simulink model "MPCFSCRL"  (R2024a)
settings: Solver=VariableStepAuto  StartTime=0.0  StopTime=0.04  RelTol=1e-3
values from neighbouring files (symbols this model uses):
  A = (2/3)*[1 -1/2 -1/2; 0 sqrt(3)/2 -sqrt(3)/2]    [AgenteRL.m]
  C = 1000e-6    (= 0.001)    [AgenteRL.m]
  Ls = 10e-3    (= 0.01)    [AgenteRL.m]
  R = 0.1    [AgenteRL.m]
  Rs = 0.1    [AgenteRL.m]
  Ts = 10e-6    (= 1e-05)    [AgenteRL.m]
  Vcc = 350    [AgenteRL.m]
  Vg = 110    [AgenteRL.m]
libraries: spsSeriesRLCBranchLib x5, spsACVoltageSourceLib x3, spsThreePhaseVIMeasurementLib x2, rllib x1, spsDCVoltageSourceLib x1, spsGroundLib x1, spsUniversalBridgeLib x1, spsVoltageMeasurementLib x1, spspowerguiLib x1
settings Model: Creator=nalv_  LastModifiedBy=Raphael Teixeira

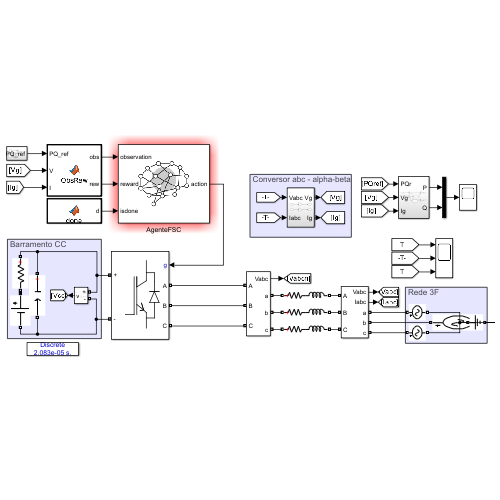
[thumbnail: Simulink's stored preview of the top-level diagram]
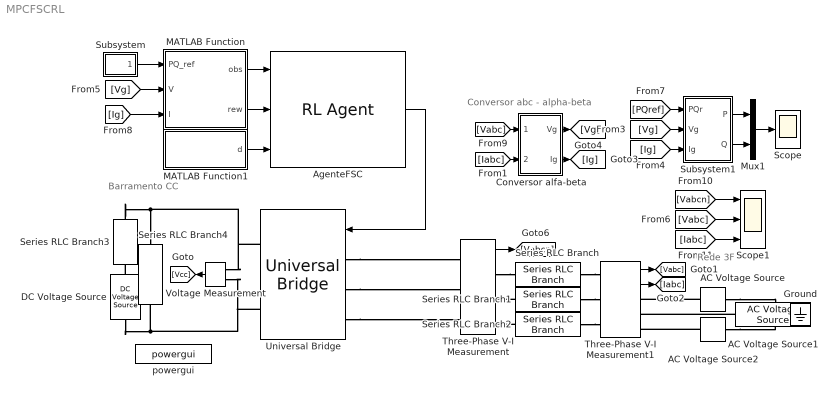
== system MPCFSCRL ==
  note: Barramento CC
  note: Conversor abc - alpha-beta
  note: Rede 3F
  AC Voltage Source : spsACVoltageSourceLib/AC Voltage Source  Amplitude=Vg  Phase=0  Frequency=60  SampleTime=Ts  Measurements=None  BusType=swing  Pref=10e3  Qref=0  Qmin=-inf  Qmax=+inf
  AC Voltage Source1 : spsACVoltageSourceLib/AC Voltage Source  Amplitude=Vg  Phase=120  Frequency=60  SampleTime=Ts  Measurements=None  BusType=swing  Pref=10e3  Qref=0  Qmin=-inf  Qmax=+inf
  AC Voltage Source2 : spsACVoltageSourceLib/AC Voltage Source  Amplitude=Vg  Phase=-120  Frequency=60  SampleTime=Ts  Measurements=None  BusType=swing  Pref=10e3  Qref=0  Qmin=-inf  Qmax=+inf
  AgenteFSC : rllib/RL Agent  Agent=agentObj  ExternalActionAsInput=off  ProvideLastAction=off  ProvideCumRwd=off  TreatAsDirectFeedthrough=on  UseStrictObservationDataTypes=off
  Conversor alfa-beta : Subsystem
  DC Voltage Source : spsDCVoltageSourceLib/DC Voltage Source  Amplitude=Vcc  Measurements=None
  Ground : spsGroundLib/Ground  LConnTagsString=a
  MATLAB Function : MATLAB Function  TreatAsAtomicUnit=on
  MATLAB Function1 : MATLAB Function  TreatAsAtomicUnit=on
  Mux1 : Mux  Inputs=2
  Scope : Scope
  Scope1 : Scope  NumInputPorts=3
  Series RLC Branch : spsSeriesRLCBranchLib/Series RLC Branch  LConnTagsString=__new0  RConnTagsString=__new0  BranchType=RL  Resistance=Rs  Inductance=Ls  SetiL0=off  InitialCurrent=0  Capacitance=1e-6  Setx0=off  InitialVoltage=0  Measurements=None
  Series RLC Branch1 : spsSeriesRLCBranchLib/Series RLC Branch  LConnTagsString=__new0  RConnTagsString=__new0  BranchType=RL  Resistance=Rs  Inductance=Ls  SetiL0=off  InitialCurrent=0  Capacitance=1e-6  Setx0=off  InitialVoltage=0  Measurements=None
  Series RLC Branch2 : spsSeriesRLCBranchLib/Series RLC Branch  LConnTagsString=__new0  RConnTagsString=__new0  BranchType=RL  Resistance=Rs  Inductance=Ls  SetiL0=off  InitialCurrent=0  Capacitance=1e-6  Setx0=off  InitialVoltage=0  Measurements=None
  Series RLC Branch3 : spsSeriesRLCBranchLib/Series RLC Branch  LConnTagsString=__new0  RConnTagsString=__new0  BranchType=R  Resistance=R  Inductance=1e-3  SetiL0=off  InitialCurrent=0  Capacitance=1e-6  Setx0=off  InitialVoltage=0  Measurements=None
  Series RLC Branch4 : spsSeriesRLCBranchLib/Series RLC Branch  LConnTagsString=__new0  RConnTagsString=__new0  BranchType=C  Resistance=1  Inductance=1e-3  SetiL0=off  InitialCurrent=0  Capacitance=C  Setx0=off  InitialVoltage=0  Measurements=None
  Subsystem : Subsystem
  Subsystem1 : Subsystem
  Three-Phase V-I Measurement : spsThreePhaseVIMeasurementLib/Three-Phase V-I Measurement  VoltageMeasurement=phase-to-ground  SetLabelV=off  LabelV=Vabc  Vpu=off  VpuLL=off  CurrentMeasurement=no  SetLabelI=off  LabelI=Iabc  Ipu=off  Pbase=100e6  Vbase=500e3  OutputType=Complex  PhasorSimulation=off  PSBequivalent=0
  Three-Phase V-I Measurement1 : spsThreePhaseVIMeasurementLib/Three-Phase V-I Measurement  VoltageMeasurement=phase-to-ground  SetLabelV=off  LabelV=Vabc  Vpu=off  VpuLL=off  CurrentMeasurement=yes  SetLabelI=off  LabelI=Iabc  Ipu=off  Pbase=100e6  Vbase=500e3  OutputType=Complex  PhasorSimulation=off  PSBequivalent=0
  Universal Bridge : spsUniversalBridgeLib/Universal Bridge  Arms=3  SnubberResistance=1e5  SnubberCapacitance=inf  Device=IGBT / Diodes  Ron=1e-3  Lon=0  ForwardVoltages="[  0  0  ]"  ForwardVoltage=0  GTOparameters=[ 10e-6 , 20e-6 ]  IGBTparameters=[ 1e-6 , 2e-6 ]  Measurements=None  Measurements_2=None  converterType=Rectifier
  Voltage Measurement : spsVoltageMeasurementLib/Voltage Measurement  PhasorSimulation=off  OutputType=Complex  PSBequivalent=0
  powergui : spspowerguiLib/powergui  Priority=1  SimulationMode=Discrete  SampleTime=Ts  frequency=60  Iterations=50  frequencyindice=60  Pbase=100e6  ErrMax=1e-4  UnitsV=kV  UnitsW=MW  buscounter=0  FunctionMessages=off  echomessages=off  EnableUseOfTLC=off  CurrentSourceSwitches=off  DisableSnubberDevices=off  DisableRonSwitches=off  DisableVfSwitches=off  DisplayEquations=off  AutomaticDiscreteSolvers=off  SolverType=Tustin/Backward Euler (TBE)  Interpol=off  ExternalGateDelay=off  methode=off  Ts=100  x0status=blocks  SPID=on  SwTol=0  HookPort=off  NonlinearTolerance=1e-4  nMaxIteration=100  ContinueOnMaxIteration=off  RestoreLinks=warning  ResistiveCurrentMeasurement=off  Frange=[0:2:500]  Ylog=off  Xlog=on  ShowGrid=off  save=off  variable=ZData  structure=0  ZoomFFT=off  StartTime=0.0  cycles=1  DisplayStyle=1  fundamental=60  FreqAxis=off  MaxFrequency=1000  frequencyindicesteady=1  RmsSteady=1  display=off
  wires:
  Conversor alfa-beta/1(Vg) -> [Vg]
  Subsystem1/1(P) -> Mux1/1
  Subsystem1/2(Q) -> Mux1/2
  Mux1/1 -> Scope/1
  Voltage Measurement/1 -> [Vcc]
  Three-Phase V-I Measurement1/1 -> [Vabc]
  [Vabc] -> Conversor alfa-beta/1(Vabc)
  Three-Phase V-I Measurement1/2 -> [Iabc]
  [Iabc] -> Conversor alfa-beta/2(Iabc)
  Conversor alfa-beta/2(Ig) -> [Ig]
  [Vg] -> Subsystem1/2(Vg)
  [Ig] -> Subsystem1/3(Ig)
  [Vg] -> MATLAB Function/2(V)
  [Ig] -> MATLAB Function/3(I)
  [PQref] -> Subsystem1/1(PQr)
  Three-Phase V-I Measurement/1 -> [Vabcn]
  [Vabcn] -> Scope1/1
  [Vabc] -> Scope1/2
  [Iabc] -> Scope1/3
  AgenteFSC/1 -> Universal Bridge/1
  Subsystem/1(PQ_ref) -> MATLAB Function/1(PQ_ref)
  MATLAB Function/1(obs) -> AgenteFSC/1
  MATLAB Function/2(rew) -> AgenteFSC/2
  MATLAB Function1/1(d) -> AgenteFSC/3
  connections:
  Universal Bridge/LConn1 -- Three-Phase V-I Measurement/LConn1
  Universal Bridge/LConn2 -- Three-Phase V-I Measurement/LConn2
  Universal Bridge/LConn3 -- Three-Phase V-I Measurement/LConn3
  Three-Phase V-I Measurement/RConn1 -- Series RLC Branch/LConn1
  Series RLC Branch1/LConn1 -- Three-Phase V-I Measurement/RConn2
  Series RLC Branch2/LConn1 -- Three-Phase V-I Measurement/RConn3
  Series RLC Branch/RConn1 -- Three-Phase V-I Measurement1/LConn1
  Series RLC Branch1/RConn1 -- Three-Phase V-I Measurement1/LConn2
  Series RLC Branch2/RConn1 -- Three-Phase V-I Measurement1/LConn3
  DC Voltage Source/RConn1 -- Series RLC Branch3/RConn1
  Series RLC Branch3/LConn1 -- Universal Bridge/RConn1 -- Voltage Measurement/LConn1 -- Series RLC Branch4/LConn1
  DC Voltage Source/LConn1 -- Universal Bridge/RConn2 -- Voltage Measurement/LConn2 -- Series RLC Branch4/RConn1
  AC Voltage Source/RConn1 -- Three-Phase V-I Measurement1/RConn1
  AC Voltage Source1/RConn1 -- Three-Phase V-I Measurement1/RConn2
  AC Voltage Source2/RConn1 -- Three-Phase V-I Measurement1/RConn3
  Ground/LConn1 -- AC Voltage Source2/LConn1 -- AC Voltage Source/LConn1 -- AC Voltage Source1/LConn1

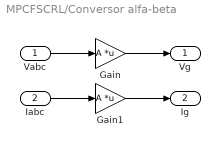
== system MPCFSCRL/Conversor alfa-beta ==
  Vabc : Inport
  Iabc : Inport  Port=2
  Gain : Gain  Gain=A  Multiplication=Matrix(K*u)
  Gain1 : Gain  Gain=A  Multiplication=Matrix(K*u)
  Vg : Outport
  Ig : Outport  Port=2
  wires:
  Vabc/1 -> Gain/1
  Gain/1 -> Vg/1
  Iabc/1 -> Gain1/1
  Gain1/1 -> Ig/1

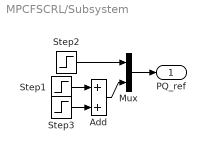
== system MPCFSCRL/Subsystem ==
  Add : Sum
  Mux : Mux  Inputs=2
  Step1 : Step  Time=0.01  Before=250  After=-250  SampleTime=Ts
  Step2 : Step  Time=0.02  Before=750  After=-750  SampleTime=Ts
  Step3 : Step  Time=0.03  After=500  SampleTime=Ts
  PQ_ref : Outport
  wires:
  Step1/1 -> Add/1
  Step2/1 -> Mux/1
  Add/1 -> Mux/2
  Step3/1 -> Add/2
  Mux/1 -> PQ_ref/1

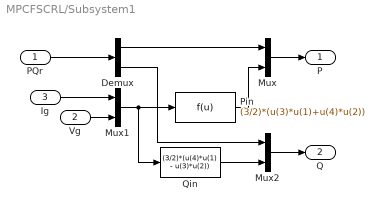
== system MPCFSCRL/Subsystem1 ==
  PQr : Inport
  Vg : Inport  Port=2
  Ig : Inport  Port=3
  Demux : Demux  Outputs=2
  Mux : Mux  Inputs=2
  Mux1 : Mux  Inputs=2
  Mux2 : Mux  Inputs=2
  Pin : Fcn  Expr=(3/2)*(u(3)*u(1)+u(4)*u(2))
  Qin : Fcn  Expr=(3/2)*(u(4)*u(1) - u(3)*u(2))
  P : Outport
  Q : Outport  Port=2
  wires:
  PQr/1 -> Demux/1
  Demux/1 -> Mux/1
  Mux/1 -> P/1
  Ig/1 -> Mux1/1
  Vg/1 -> Mux1/2
  Mux1/1 -> Qin/1, Pin/1
  Pin/1 -> Mux/2
  Qin/1 -> Mux2/2
  Demux/2 -> Mux2/1
  Mux2/1 -> Q/1

== matlab function MPCFSCRL/MATLAB Function1 ==
  data: d output
function d = done()
    % Obtém o tempo atual da simulação no Simulink
    sim_time = get_param(bdroot, 'SimulationTime');

    % Definição do tempo máximo do episódio
    max_time = 0.04;  % Tempo limite para o episódio (40ms)

    % Condição para encerrar o episódio
    if sim_time >= max_time
        d = 1;  % O episódio terminou
    else
        d = 0;  % O episódio continua
    end
end

== matlab function MPCFSCRL/MATLAB Function ==
  data: PQ_ref input; obs output; V input; I input; rew output
function [obs, rew] = ObsRew(PQ_ref, V, I)
    % Definição dos pesos para a minimização dos erros de potência
    w_P = 1.0;  % Peso do erro de potência ativa
    w_Q = 1.0;  % Peso do erro de potência reativa

    % Extração das referências de potência ativa e reativa
    P_ref = PQ_ref(1);
    Q_ref = PQ_ref(2);

    % Extração das componentes alpha e beta das tensões e correntes
    V_alpha = V(1);
    V_beta  = V(2);
    I_alpha = I(1);
    I_beta  = I(2);

    % Cálculo da potência ativa e reativa medida
    P = V_alpha * I_alpha + V_beta * I_beta;  % Potência ativa real
    Q = V_beta * I_alpha - V_alpha * I_beta;  % Potência reativa real

    % Cálculo dos erros de potência
    e_P = P_ref - P;
    e_Q = Q_ref - Q;

    % Cálculo da recompensa (quanto menor o erro, maior a recompensa)
    rew = exp(- (w_P * e_P^2 + w_Q * e_Q^2));

    % Agrupamento das variáveis de estado em um único vetor de saída (observação)
    obs = [P_ref, Q_ref, V_alpha, V_beta, I_alpha, I_beta];
end
